simulink model "PMLSM_ControlCore_Block"  (R2026a)
settings: Solver=FixedStepDiscrete  StopTime=1  FixedStep=1e-4
values from neighbouring files (symbols this model uses):
  CPU_Clock = 200e6    (= 200000000)    [PMSLM_Init_Params_MBDL4.m]
  Current_Control_Mode = 2    [init_PMLSM_mil_test_params.m]
  DeadTime_Comp_Enable = 0    [init_PMLSM_mil_test_params.m]
  delay_N = 50    [PMSLM_Init_Params_MBDL4.m]
  DPCC_Ld_Factor = 1    [init_PMLSM_mil_test_params.m]
  DPCC_Lq_Factor = 1    [init_PMLSM_mil_test_params.m]
  DPCC_Psi_Factor = 1    [init_PMLSM_mil_test_params.m]
  DPCC_Rs_Factor = 1    [init_PMLSM_mil_test_params.m]
  DPICC_Ld_Factor = 1    [init_PMLSM_mil_test_params.m]
  DPICC_Lq_Factor = 1    [init_PMLSM_mil_test_params.m]
  Hold_Ticks = 30000    [PMSLM_Init_Params_MBDL4.m]
  Id_Init_Step = Id_Init_Target / Ramp_Ticks    (= 5e-05)    [PMSLM_Init_Params_MBDL4.m]
  Id_Init_Target = 0.5    [PMSLM_Init_Params_MBDL4.m]
  Id_Release_Ramp_Ticks = 2000    [PMSLM_Init_Params_MBDL4.m]
  Iq_fric_run = 0.05    [PMSLM_Init_Params_MBDL4.m]
  Iq_fric_start = 0.40    (= 0.4)    [PMSLM_Init_Params_MBDL4.m]
  Iq_int_limit = 0.10    (= 0.1)    [PMSLM_Init_Params_MBDL4.m]
  Kaw_d = Kaw_q    (= 0.2)    [PMSLM_Init_Params_MBDL4.m]
  Kaw_q = 0.2    [PMSLM_Init_Params_MBDL4.m]
  Kaw_s = 0.4    [PMSLM_Init_Params_MBDL4.m]
  Ki_ACR = ACR_Commissioning_Scale*Ki_ACR_Baseline    (= 2962.5)    [PMSLM_Init_Params_MBDL4.m]    (also in init_PMLSM_mil_test_params.m = Kp_ACR*PMLSM_Rs_ohm/PMLSM_Lq_H)
  Ki_ASR = 0.05    [PMSLM_Init_Params_MBDL4.m]
  Kp_ACR = ACR_Commissioning_Scale*Kp_ACR_Baseline    (= 2.18125)    [PMSLM_Init_Params_MBDL4.m]    (also in init_PMLSM_mil_test_params.m = PMLSM_Lq_H/(4*MIL_AUM3S4_Current_PI_xi^2*MIL_AUM3S4_Current_)
  Kp_ASR = 0.03    [PMSLM_Init_Params_MBDL4.m]
  Kp_pos = 5    [PMSLM_Init_Params_MBDL4.m]
  PICDO_Dhat_Limit_A = 3.0    (= 3)    [init_PMLSM_mil_test_params.m]
  PICDO_Kd = 0.25    [init_PMLSM_mil_test_params.m]
  PICDO_Kx = 1.0    (= 1)    [init_PMLSM_mil_test_params.m]
  PMLSM_deadtime_ratio = PMLSM_deadtime_s * PMLSM_pwm_freq_Hz    (= 0.01)    [init_PMLSM_plant_params.m]
  PMLSM_Ld_H = Ld    (= 0.001745)    [PMSLM_Init_Params_MBDL4.m]    (also in init_PMLSM_plant_params.m)
  PMLSM_Lq_H = Lq    (= 0.001745)    [PMSLM_Init_Params_MBDL4.m]    (also in init_PMLSM_plant_params.m)
  PMLSM_psi_f_Wb = flux    (= 0.141)    [PMSLM_Init_Params_MBDL4.m]    (also in init_PMLSM_plant_params.m)
  PMLSM_Rs_ohm = Rs    (= 2.37)    [PMSLM_Init_Params_MBDL4.m]    (also in init_PMLSM_plant_params.m)
  Pos_deadband = 0.02    [PMSLM_Init_Params_MBDL4.m]
  Ramp_Ticks = 10000    [PMSLM_Init_Params_MBDL4.m]
  Speed_Feedback_Mode = 1    [init_PMLSM_mil_test_params.m]
  Speed_loop_Iq_Limit = Iq_Limit    (= 0.3)    [PMSLM_Init_Params_MBDL4.m]
  Tau_e_mm = 60    [PMSLM_Init_Params_MBDL4.m]
  theta_align_const = 0    [PMSLM_Init_Params_MBDL4.m]
  Theta_Offset_Fine = Simulink.Parameter    [PMSLM_Init_Params_MBDL4.m]
  Ts = 1 / PWM_Freq    (= 0.0001)    [PMSLM_Init_Params_MBDL4.m]
  Ts_ACR = 1e-4    (= 0.0001)    [PMSLM_Init_Params_MBDL4.m]
  Ts_ASR = 1e-3    (= 0.001)    [PMSLM_Init_Params_MBDL4.m]
  Ts_DPICC = 1e-4    (= 0.0001)    [init_PMLSM_mil_test_params.m]
  Udc = 48    [PMSLM_Init_Params_MBDL4.m]    (also in init_PMLSM_mil_test_params.m)
  Uq_Zero_EN = 0：q 轴用正常 PI    [PMSLM_Init_Params_MBDL4.m]
  v_ff_eps = 0.5    [PMSLM_Init_Params_MBDL4.m]
  V_meas_max = 500    [PMSLM_Init_Params_MBDL4.m]
  v_meas_zero_eps = 0.5    [PMSLM_Init_Params_MBDL4.m]
  v_over_eps = 3    [PMSLM_Init_Params_MBDL4.m]
  V_pos_max_mmps = 10    [PMSLM_Init_Params_MBDL4.m]
  v_ref_max = 20    [PMSLM_Init_Params_MBDL4.m]
  v_ref_set_step_dn = v_ref_set_rate_dn * Ts    (= 0.005)    [PMSLM_Init_Params_MBDL4.m]
  v_ref_set_step_up = v_ref_set_rate_up * Ts    (= 0.005)    [PMSLM_Init_Params_MBDL4.m]
  v_ref_zero_eps = 0.2    [PMSLM_Init_Params_MBDL4.m]
  v_stick_off = 3.0    (= 3)    [PMSLM_Init_Params_MBDL4.m]
  v_stick_on = 1.0    (= 1)    [PMSLM_Init_Params_MBDL4.m]
  X_max_hard = 500    [PMSLM_Init_Params_MBDL4.m]
  X_max_soft = 470    [PMSLM_Init_Params_MBDL4.m]
  X_min_hard = -500    [PMSLM_Init_Params_MBDL4.m]
  X_min_soft = -470    [PMSLM_Init_Params_MBDL4.m]
libraries: hdlsllib x13, simulink x11, mcbeeMathTransformLib x2, mcbcontrolslib x1
(part 2 of 3)

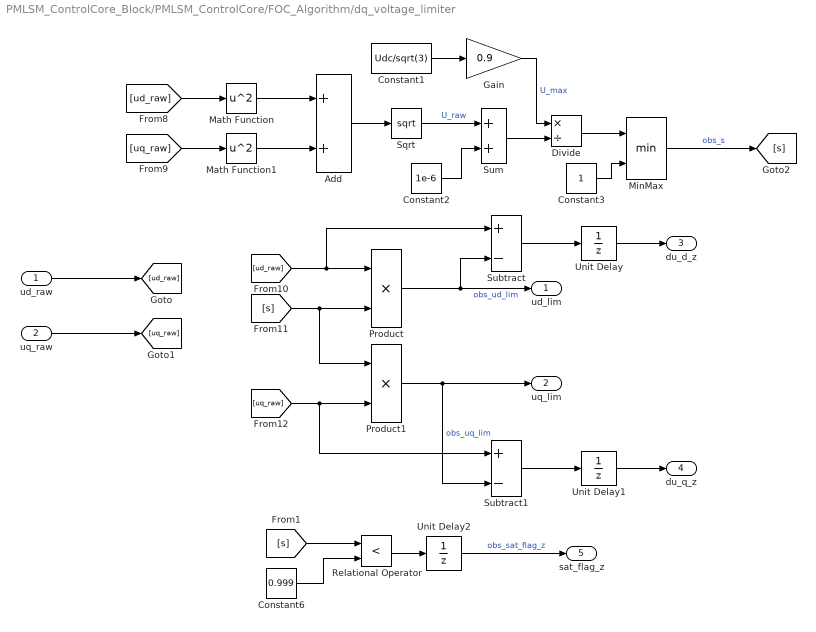
== system PMLSM_ControlCore_Block/PMLSM_ControlCore/FOC_Algorithm/dq_voltage_limiter ==
  ud_raw : Inport
  uq_raw : Inport  Port=2
  Add : Sum
  Constant1 : Constant  Value=Udc/sqrt(3)  OutDataTypeStr=double
  Constant2 : Constant  Value=1e-6  OutDataTypeStr=double
  Constant3 : Constant  OutDataTypeStr=double
  Constant6 : Constant  Value=0.999
  Divide : Product  Inputs=*/  OutDataTypeStr=double
  Gain : Gain  Gain=0.9  OutDataTypeStr=double
  Math Function : Math  Operator=square
  Math Function1 : Math  Operator=square
  MinMax : MinMax  Inputs=2
  Product : Product
  Product1 : Product  OutDataTypeStr=double
  Relational Operator : RelationalOperator  Operator=<  OutDataTypeStr=boolean  RndMeth=Simplest  InputSameDT=off
  Sqrt : Sqrt
  Subtract : Sum  Inputs=+-
  Subtract1 : Sum  Inputs=+-
  Sum : Sum
  Unit Delay : UnitDelay  SampleTime=-1
  Unit Delay1 : UnitDelay  SampleTime=-1
  Unit Delay2 : UnitDelay  SampleTime=-1
  ud_lim : Outport
  uq_lim : Outport  Port=2
  du_d_z : Outport  Port=3
  du_q_z : Outport  Port=4
  sat_flag_z : Outport  Port=5
  wires:
  Unit Delay2/1 -> sat_flag_z/1  "obs_sat_flag_z"
  Relational Operator/1 -> Unit Delay2/1
  [s] -> Relational Operator/1
  Constant6/1 -> Relational Operator/2
  Unit Delay1/1 -> du_q_z/1
  Unit Delay/1 -> du_d_z/1
  uq_raw/1 -> [uq_raw]
  ud_raw/1 -> [ud_raw]
  Subtract1/1 -> Unit Delay1/1
  Subtract/1 -> Unit Delay/1
  [uq_raw] -> Product1/2, Subtract1/1
  Product/1 -> ud_lim/1, Subtract/2  "obs_ud_lim"
  [ud_raw] -> Product/1, Subtract/1
  [s] -> Product/2, Product1/1
  Product1/1 -> Subtract1/2, uq_lim/1  "obs_uq_lim"
  MinMax/1 -> [s]  "obs_s"
  [ud_raw] -> Math Function/1
  [uq_raw] -> Math Function1/1
  Math Function/1 -> Add/1
  Math Function1/1 -> Add/2
  Sqrt/1 -> Sum/1  "U_raw"
  Gain/1 -> Divide/1  "U_max"
  Divide/1 -> MinMax/1
  Constant1/1 -> Gain/1
  Add/1 -> Sqrt/1
  Constant3/1 -> MinMax/2
  Constant2/1 -> Sum/2
  Sum/1 -> Divide/2

== system PMLSM_ControlCore_Block/PMLSM_ControlCore/Reference_Manager/v_ref_set_slew_limiter ==
  v_ref_set : Inport
  Add : Sum
  Saturation : Saturate  UpperLimit=v_ref_set_step_up  LowerLimit=-v_ref_set_step_dn
  Subtract : Sum  Inputs=+-
  v_ref_set_lim_z : UnitDelay  SampleTime=-1
  v_ref_set_limited : Outport
  wires:
  Add/1 -> v_ref_set_lim_z/1, v_ref_set_limited/1
  Subtract/1 -> Saturation/1
  Saturation/1 -> Add/1
  v_ref_set/1 -> Subtract/1
  v_ref_set_lim_z/1 -> Subtract/2, Add/2

== system PMLSM_ControlCore_Block/PMLSM_ControlCore/Triggered_Speed_loop/friction_compensation ==
  note: if start_mode == 1
      | 	iq_fric_mag = Iq_fric_start;
      | else
      | 	iq_fric_mag = Iq_fric_run;
      |
      | if ff_enable
      | 	iq_ff = iq_fric_mag * sign(v_ref);
      |  else
      | 	iq_ff = 0;
  v_ref : Inport
  abs_v_ref : Inport  Port=2
  abs_v_mmps : Inport  Port=3
  e_v : Inport  Port=4
  Compare To Constant1 : simulink/Logic and Bit Operations/Compare To Constant  relop=>  const=-v_over_eps  OutDataTypeStr=boolean
  Compare To Constant2 : simulink/Logic and Bit Operations/Compare To Constant  relop=>  const=v_ff_eps  OutDataTypeStr=boolean
  Constant1 : Constant  Value=Iq_fric_start
  Constant5 : Constant  Value=0
  Constant6 : Constant  Value=Iq_fric_run
  Gain : Gain  Gain=-1
  Logical Operator : Logic  AllPortsSameDT=off  OutDataTypeStr=boolean
  Product : Product
  Product1 : Product
  Product2 : Product
  Relay : Relay  OnSwitchValue=-v_stick_on  OffSwitchValue=-v_stick_off
  Sign : Signum
  Sign1 : Signum
  Switch : Switch  Criteria=u2 > Threshold  Threshold=0.5  SaturateOnIntegerOverflow=off  InputSameDT=off
  Switch2 : Switch  Criteria=u2 > Threshold  Threshold=0.5  SaturateOnIntegerOverflow=off  InputSameDT=off
  iq_ff : Outport
  wires:
  Gain/1 -> Relay/1
  Relay/1 -> Switch/2  "fric_start_mode"
  abs_v_mmps/1 -> Gain/1
  Logical Operator/1 -> Switch2/2  "ff_enable"
  Compare To Constant1/1 -> Logical Operator/2
  Compare To Constant2/1 -> Logical Operator/1
  Product2/1 -> Compare To Constant1/1
  e_v/1 -> Product2/2
  Product1/1 -> Switch/1
  Constant1/1 -> Product1/2
  Sign1/1 -> Product1/1
  Product/1 -> Switch/3
  Switch/1 -> Switch2/1
  Switch2/1 -> iq_ff/1  "iq_ff"
  abs_v_ref/1 -> Compare To Constant2/1
  Constant6/1 -> Product/2
  Constant5/1 -> Switch2/3
  Sign/1 -> Product/1, Product2/1
  v_ref/1 -> Sign1/1, Sign/1

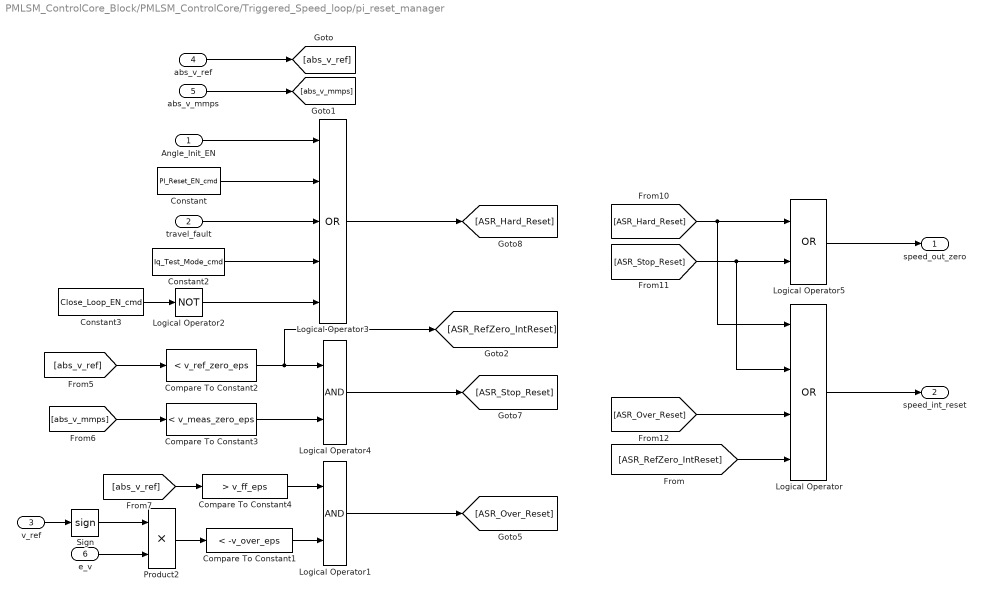
== system PMLSM_ControlCore_Block/PMLSM_ControlCore/Triggered_Speed_loop/pi_reset_manager ==
  Angle_Init_EN : Inport
  travel_fault : Inport  Port=2
  v_ref : Inport  Port=3
  abs_v_ref : Inport  Port=4
  abs_v_mmps : Inport  Port=5
  e_v : Inport  Port=6
  Compare To Constant1 : simulink/Logic and Bit Operations/Compare To Constant  relop=<  const=-v_over_eps  OutDataTypeStr=boolean
  Compare To Constant2 : simulink/Logic and Bit Operations/Compare To Constant  relop=<  const=v_ref_zero_eps  OutDataTypeStr=boolean
  Compare To Constant3 : simulink/Logic and Bit Operations/Compare To Constant  relop=<  const=v_meas_zero_eps  OutDataTypeStr=boolean
  Compare To Constant4 : simulink/Logic and Bit Operations/Compare To Constant  relop=>  const=v_ff_eps  OutDataTypeStr=boolean
  Constant : DataStoreRead  DataStoreName=PI_Reset_EN_cmd  IndexOptions=Index vector (dialog)  Indices=1  OutputSizes=1
  Constant2 : DataStoreRead  DataStoreName=Iq_Test_Mode_cmd  IndexOptions=Index vector (dialog)  Indices=1  OutputSizes=1
  Constant3 : DataStoreRead  DataStoreName=Close_Loop_EN_cmd  IndexOptions=Index vector (dialog)  Indices=1  OutputSizes=1
  Logical Operator : Logic  Operator=OR  Inputs=4  AllPortsSameDT=off  OutDataTypeStr=boolean
  Logical Operator1 : Logic  AllPortsSameDT=off  OutDataTypeStr=boolean
  Logical Operator2 : Logic  Operator=NOT  AllPortsSameDT=off  OutDataTypeStr=boolean
  Logical Operator3 : Logic  Operator=OR  Inputs=5  AllPortsSameDT=off  OutDataTypeStr=boolean
  Logical Operator4 : Logic  AllPortsSameDT=off  OutDataTypeStr=boolean
  Logical Operator5 : Logic  Operator=OR  AllPortsSameDT=off  OutDataTypeStr=boolean
  Product2 : Product
  Sign : Signum
  speed_out_zero : Outport
  speed_int_reset : Outport  Port=2
  wires:
  [ASR_RefZero_IntReset] -> Logical Operator/4
  Logical Operator1/1 -> [ASR_Over_Reset]
  Logical Operator/1 -> speed_int_reset/1
  [ASR_Over_Reset] -> Logical Operator/3
  [ASR_Hard_Reset] -> Logical Operator/1, Logical Operator5/1
  [ASR_Stop_Reset] -> Logical Operator/2, Logical Operator5/2
  Logical Operator4/1 -> [ASR_Stop_Reset]
  Logical Operator5/1 -> speed_out_zero/1
  Logical Operator3/1 -> [ASR_Hard_Reset]
  Compare To Constant3/1 -> Logical Operator4/2
  abs_v_mmps/1 -> [abs_v_mmps]
  abs_v_ref/1 -> [abs_v_ref]
  v_ref/1 -> Sign/1
  Angle_Init_EN/1 -> Logical Operator3/1
  Compare To Constant4/1 -> Logical Operator1/1
  Compare To Constant1/1 -> Logical Operator1/2
  Product2/1 -> Compare To Constant1/1
  Sign/1 -> Product2/1
  travel_fault/1 -> Logical Operator3/3
  e_v/1 -> Product2/2
  [abs_v_ref] -> Compare To Constant4/1
  [abs_v_mmps] -> Compare To Constant3/1
  Logical Operator2/1 -> Logical Operator3/5
  [abs_v_ref] -> Compare To Constant2/1
  Compare To Constant2/1 -> Logical Operator4/1, [ASR_RefZero_IntReset]
  Constant2/1 -> Logical Operator3/4
  Constant3/1 -> Logical Operator2/1
  Constant/1 -> Logical Operator3/2

== system PMLSM_ControlCore_Block/PMLSM_ControlCore/FOC_Algorithm/DPCC_Current_Controller/DPCC_DPICC_Select ==
  ud_dpcc : Inport
  uq_dpcc : Inport  Port=2
  ud_dpicc : Inport  Port=3
  uq_dpicc : Inport  Port=4
  dpicc_active : Inport  Port=5
  Current_Control_Mode : Inport  Port=6
  ud_pi : Inport  Port=7
  uq_pi : Inport  Port=8
  d_active_select : Switch  Threshold=0.5
  d_mode_select : Switch  Threshold=2.5
  q_active_select : Switch  Threshold=0.5
  q_mode_select : Switch  Threshold=2.5
  ud_selected : Outport
  uq_selected : Outport  Port=2
  wires:
  q_mode_select/1 -> uq_selected/1
  d_mode_select/1 -> ud_selected/1
  uq_dpcc/1 -> q_mode_select/3
  q_active_select/1 -> q_mode_select/1
  ud_dpcc/1 -> d_mode_select/3
  Current_Control_Mode/1 -> q_mode_select/2, d_mode_select/2
  d_active_select/1 -> d_mode_select/1
  uq_pi/1 -> q_active_select/3
  uq_dpicc/1 -> q_active_select/1
  ud_pi/1 -> d_active_select/3
  dpicc_active/1 -> d_active_select/2, q_active_select/2
  ud_dpicc/1 -> d_active_select/1

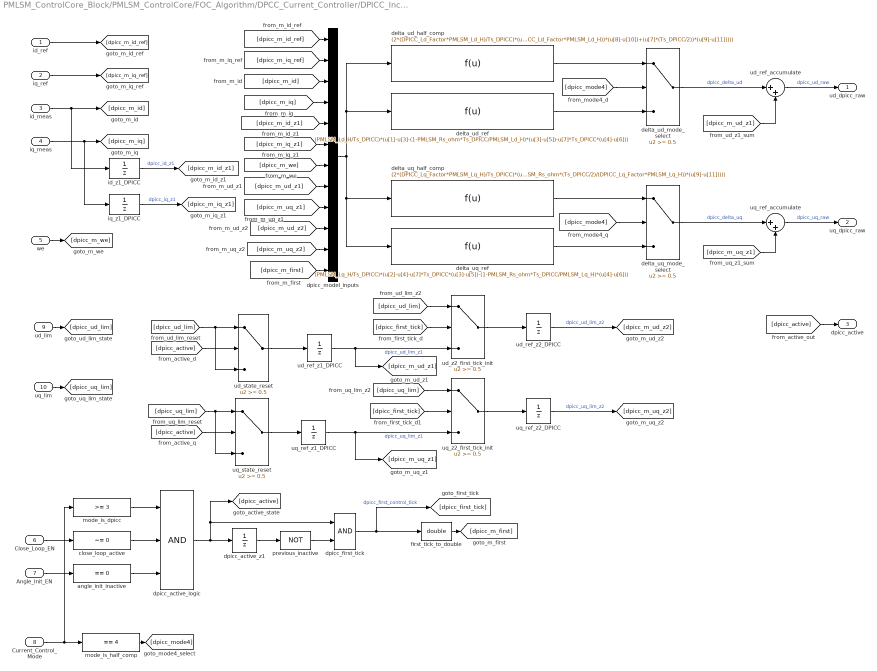
== system PMLSM_ControlCore_Block/PMLSM_ControlCore/FOC_Algorithm/DPCC_Current_Controller/DPICC_Incremental_Core ==
  id_ref : Inport
  iq_ref : Inport  Port=2
  id_meas : Inport  Port=3
  iq_meas : Inport  Port=4
  we : Inport  Port=5
  Close_Loop_EN : Inport  Port=6
  Angle_Init_EN : Inport  Port=7
  Current_Control_Mode : Inport  Port=8
  ud_lim : Inport  Port=9
  uq_lim : Inport  Port=10
  angle_init_inactive : hdlsllib/Logic and Bit Operations/Compare To Constant  relop===  const=0  OutDataTypeStr=boolean
  close_loop_active : hdlsllib/Logic and Bit Operations/Compare To Constant  relop=~=  const=0  OutDataTypeStr=boolean
  delta_ud_half_comp : Fcn  Expr=(2*(DPICC_Ld_Factor*PMLSM_Ld_H)/Ts_DPICC)*(u[1]-u[3]-(1-u[12])*(((1-PMLSM_Rs_ohm*(Ts_DPICC/2)/(DPICC_Ld_Factor*PMLSM_Ld_H))^2-(u[7]*(Ts_DPICC/2))^2)*(u[3]-u[5])+2*(1-PMLSM_Rs_ohm*(Ts_DPICC/2)/(DPICC_Ld_Factor*PMLSM_Ld_H))*(u[7]*(Ts_DPICC/2))*(u[4]-u[6])+(Ts_DPICC/2/(DPICC_Ld_Factor*PMLSM_Ld_H))*((1-PMLSM_Rs_ohm*(Ts_DPICC/2)/(DPICC_Ld_Factor*PMLSM_Ld_H))*(u[8]-u[10])+(u[7]*(Ts_DPICC/2))*(u[9]-u[11]))))
  delta_ud_mode_select : Switch  Threshold=0.5
  delta_ud_ref : Fcn  Expr=(PMLSM_Ld_H/Ts_DPICC)*(u[1]-u[3]-(1-PMLSM_Rs_ohm*Ts_DPICC/PMLSM_Ld_H)*(u[3]-u[5])-u[7]*Ts_DPICC*(u[4]-u[6]))
  delta_uq_half_comp : Fcn  Expr=(2*(DPICC_Lq_Factor*PMLSM_Lq_H)/Ts_DPICC)*(u[2]-u[4]-(1-u[12])*(-2*(1-PMLSM_Rs_ohm*(Ts_DPICC/2)/(DPICC_Lq_Factor*PMLSM_Lq_H))*(u[7]*(Ts_DPICC/2))*(u[3]-u[5])+((1-PMLSM_Rs_ohm*(Ts_DPICC/2)/(DPICC_Lq_Factor*PMLSM_Lq_H))^2-(u[7]*(Ts_DPICC/2))^2)*(u[4]-u[6])+(Ts_DPICC/2/(DPICC_Lq_Factor*PMLSM_Lq_H))*(-(u[7]*(Ts_DPICC/2))*(u[8]-u[10])+(1-PMLSM_Rs_ohm*(Ts_DPICC/2)/(DPICC_Lq_Factor*PMLSM_Lq_H))*(u[9]-u[11]))))
  delta_uq_mode_select : Switch  Threshold=0.5
  delta_uq_ref : Fcn  Expr=(PMLSM_Lq_H/Ts_DPICC)*(u[2]-u[4]-u[7]*Ts_DPICC*(u[3]-u[5])-(1-PMLSM_Rs_ohm*Ts_DPICC/PMLSM_Lq_H)*(u[4]-u[6]))
  dpicc_active_logic : Logic  Inputs=3
  dpicc_active_z1 : UnitDelay  SampleTime=-1
  dpicc_first_tick : Logic
  dpicc_model_inputs : Mux  Inputs=12
  first_tick_to_double : DataTypeConversion  OutDataTypeStr=double
  id_z1_DPICC : UnitDelay  SampleTime=-1  StateName=id_z1_DPICC
  iq_z1_DPICC : UnitDelay  SampleTime=-1  StateName=iq_z1_DPICC
  mode_is_dpicc : hdlsllib/Logic and Bit Operations/Compare To Constant  relop=>=  const=3  OutDataTypeStr=boolean
  mode_is_half_comp : hdlsllib/Logic and Bit Operations/Compare To Constant  relop===  const=4  OutDataTypeStr=boolean
  previous_inactive : Logic  Operator=NOT  Inputs=1
  ud_ref_accumulate : Sum  Inputs=|++
  ud_ref_z1_DPICC : UnitDelay  SampleTime=-1  StateName=ud_ref_z1_DPICC
  ud_ref_z2_DPICC : UnitDelay  SampleTime=-1
  ud_state_reset : Switch  Threshold=0.5
  ud_z2_first_tick_init : Switch  Threshold=0.5
  uq_ref_accumulate : Sum  Inputs=|++
  uq_ref_z1_DPICC : UnitDelay  SampleTime=-1  StateName=uq_ref_z1_DPICC
  uq_ref_z2_DPICC : UnitDelay  SampleTime=-1
  uq_state_reset : Switch  Threshold=0.5
  uq_z2_first_tick_init : Switch  Threshold=0.5
  ud_dpicc_raw : Outport
  uq_dpicc_raw : Outport  Port=2
  dpicc_active : Outport  Port=3
  wires:
  uq_ref_accumulate/1 -> uq_dpicc_raw/1  "dpicc_uq_raw"
  ud_ref_accumulate/1 -> ud_dpicc_raw/1  "dpicc_ud_raw"
  uq_ref_z1_DPICC/1 -> [dpicc_m_uq_z1], uq_z2_first_tick_init/3  "dpicc_uq_lim_z1"
  delta_uq_ref/1 -> delta_uq_mode_select/3
  ud_ref_z1_DPICC/1 -> [dpicc_m_ud_z1], ud_z2_first_tick_init/3  "dpicc_ud_lim_z1"
  delta_ud_ref/1 -> delta_ud_mode_select/3
  uq_state_reset/1 -> uq_ref_z1_DPICC/1
  ud_state_reset/1 -> ud_ref_z1_DPICC/1
  uq_lim/1 -> [dpicc_uq_lim]
  ud_lim/1 -> [dpicc_ud_lim]
  dpicc_model_inputs/1 -> delta_uq_half_comp/1, delta_uq_ref/1, delta_ud_half_comp/1, delta_ud_ref/1
  we/1 -> [dpicc_m_we]
  iq_z1_DPICC/1 -> [dpicc_m_iq_z1]  "dpicc_iq_z1"
  id_z1_DPICC/1 -> [dpicc_m_id_z1]  "dpicc_id_z1"
  iq_ref/1 -> [dpicc_m_iq_ref]
  id_ref/1 -> [dpicc_m_id_ref]
  iq_meas/1 -> [dpicc_m_iq], iq_z1_DPICC/1
  id_meas/1 -> [dpicc_m_id], id_z1_DPICC/1
  Current_Control_Mode/1 -> mode_is_half_comp/1, mode_is_dpicc/1
  Close_Loop_EN/1 -> close_loop_active/1
  Angle_Init_EN/1 -> angle_init_inactive/1
  mode_is_dpicc/1 -> dpicc_active_logic/1
  close_loop_active/1 -> dpicc_active_logic/2
  angle_init_inactive/1 -> dpicc_active_logic/3
  dpicc_active_logic/1 -> dpicc_first_tick/1, [dpicc_active], dpicc_active_z1/1
  dpicc_active_z1/1 -> previous_inactive/1
  previous_inactive/1 -> dpicc_first_tick/2
  delta_ud_half_comp/1 -> delta_ud_mode_select/1
  mode_is_half_comp/1 -> [dpicc_mode4]
  delta_uq_half_comp/1 -> delta_uq_mode_select/1
  delta_ud_mode_select/1 -> ud_ref_accumulate/1  "dpicc_delta_ud"
  delta_uq_mode_select/1 -> uq_ref_accumulate/1  "dpicc_delta_uq"
  dpicc_first_tick/1 -> first_tick_to_double/1, [dpicc_first_tick]  "dpicc_first_control_tick"
  ud_z2_first_tick_init/1 -> ud_ref_z2_DPICC/1
  ud_ref_z2_DPICC/1 -> [dpicc_m_ud_z2]  "dpicc_ud_lim_z2"
  uq_z2_first_tick_init/1 -> uq_ref_z2_DPICC/1
  uq_ref_z2_DPICC/1 -> [dpicc_m_uq_z2]  "dpicc_uq_lim_z2"
  first_tick_to_double/1 -> [dpicc_m_first]
  [dpicc_m_id_ref] -> dpicc_model_inputs/1
  [dpicc_m_iq_ref] -> dpicc_model_inputs/2
  [dpicc_m_id] -> dpicc_model_inputs/3
  [dpicc_m_iq] -> dpicc_model_inputs/4
  [dpicc_m_id_z1] -> dpicc_model_inputs/5
  [dpicc_m_iq_z1] -> dpicc_model_inputs/6
  [dpicc_m_we] -> dpicc_model_inputs/7
  [dpicc_m_ud_z1] -> dpicc_model_inputs/8
  [dpicc_m_uq_z1] -> dpicc_model_inputs/9
  [dpicc_m_ud_z2] -> dpicc_model_inputs/10
  [dpicc_m_uq_z2] -> dpicc_model_inputs/11
  [dpicc_m_first] -> dpicc_model_inputs/12
  [dpicc_mode4] -> delta_ud_mode_select/2
  [dpicc_mode4] -> delta_uq_mode_select/2
  [dpicc_first_tick] -> ud_z2_first_tick_init/2
  [dpicc_first_tick] -> uq_z2_first_tick_init/2
  [dpicc_active] -> ud_state_reset/2
  [dpicc_active] -> uq_state_reset/2
  [dpicc_active] -> dpicc_active/1
  [dpicc_ud_lim] -> ud_state_reset/1, ud_state_reset/3
  [dpicc_ud_lim] -> ud_z2_first_tick_init/1
  [dpicc_uq_lim] -> uq_state_reset/3, uq_state_reset/1
  [dpicc_uq_lim] -> uq_z2_first_tick_init/1
  [dpicc_m_ud_z1] -> ud_ref_accumulate/2
  [dpicc_m_uq_z1] -> uq_ref_accumulate/2

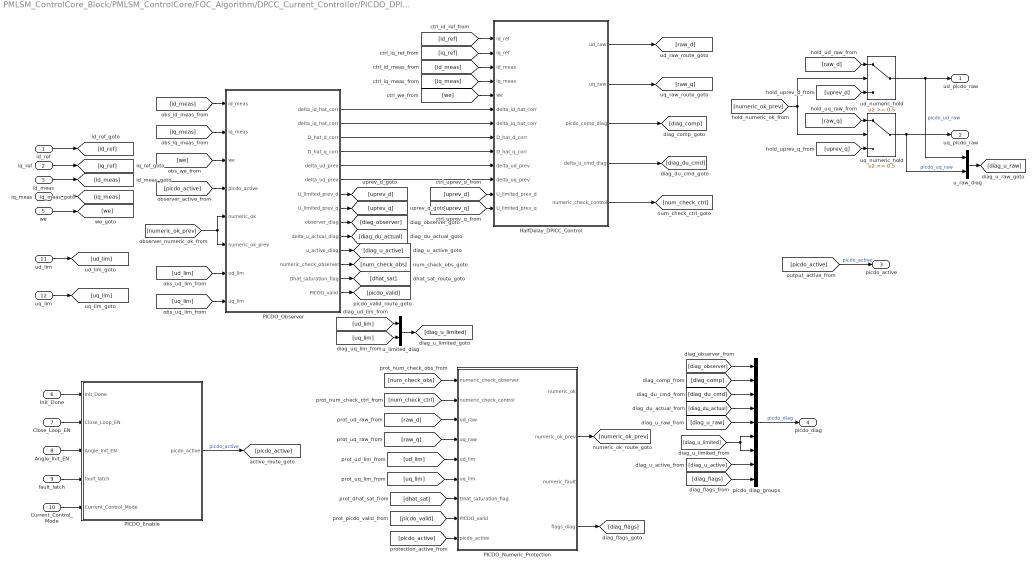
== system PMLSM_ControlCore_Block/PMLSM_ControlCore/FOC_Algorithm/DPCC_Current_Controller/PICDO_DPICC_Core ==
  id_ref : Inport
  iq_ref : Inport  Port=2
  id_meas : Inport  Port=3
  iq_meas : Inport  Port=4
  we : Inport  Port=5
  Init_Done : Inport  Port=6
  Close_Loop_EN : Inport  Port=7
  Angle_Init_EN : Inport  Port=8
  fault_latch : Inport  Port=9
  Current_Control_Mode : Inport  Port=10
  ud_lim : Inport  Port=11
  uq_lim : Inport  Port=12
  HalfDelay_DPICC_Control : Subsystem
  PICDO_Enable : Subsystem
  PICDO_Numeric_Protection : Subsystem
  PICDO_Observer : Subsystem
  picdo_diag_groups : Mux  Inputs=9
  u_limited_diag : Mux  Inputs=2
  u_raw_diag : Mux  Inputs=2
  ud_numeric_hold : Switch  Threshold=0.5
  uq_numeric_hold : Switch  Threshold=0.5
  ud_picdo_raw : Outport
  uq_picdo_raw : Outport  Port=2
  picdo_active : Outport  Port=3
  picdo_diag : Outport  Port=4
  wires:
  [numeric_ok_prev] -> uq_numeric_hold/2, ud_numeric_hold/2
  [numeric_ok_prev] -> PICDO_Observer/5(numeric_ok), PICDO_Observer/6(numeric_ok_prev)
  PICDO_Numeric_Protection/2(numeric_ok_prev) -> [numeric_ok_prev]
  [picdo_active] -> picdo_active/1  "picdo_active"
  [picdo_active] -> PICDO_Numeric_Protection/9(picdo_active)
  [picdo_active] -> PICDO_Observer/4(picdo_active)
  PICDO_Enable/1(picdo_active) -> [picdo_active]  "picdo_active"
  Init_Done/1 -> PICDO_Enable/1(Init_Done)
  Close_Loop_EN/1 -> PICDO_Enable/2(Close_Loop_EN)
  Angle_Init_EN/1 -> PICDO_Enable/3(Angle_Init_EN)
  fault_latch/1 -> PICDO_Enable/4(fault_latch)
  Current_Control_Mode/1 -> PICDO_Enable/5(Current_Control_Mode)
  id_meas/1 -> [id_meas]
  iq_meas/1 -> [iq_meas]
  we/1 -> [we]
  ud_lim/1 -> [ud_lim]
  uq_lim/1 -> [uq_lim]
  id_ref/1 -> [id_ref]
  iq_ref/1 -> [iq_ref]
  PICDO_Observer/1(delta_id_hat_corr) -> HalfDelay_DPICC_Control/6(delta_id_hat_corr)
  PICDO_Observer/2(delta_iq_hat_corr) -> HalfDelay_DPICC_Control/7(delta_iq_hat_corr)
  PICDO_Observer/3(D_hat_d_corr) -> HalfDelay_DPICC_Control/8(D_hat_d_corr)
  PICDO_Observer/4(D_hat_q_corr) -> HalfDelay_DPICC_Control/9(D_hat_q_corr)
  PICDO_Observer/5(delta_ud_prev) -> HalfDelay_DPICC_Control/10(delta_ud_prev)
  PICDO_Observer/6(delta_uq_prev) -> HalfDelay_DPICC_Control/11(delta_uq_prev)
  PICDO_Observer/7(U_limited_prev_d) -> [uprev_d]
  PICDO_Observer/8(U_limited_prev_q) -> [uprev_q]
  ud_numeric_hold/1 -> u_raw_diag/1, ud_picdo_raw/1  "picdo_ud_raw"
  uq_numeric_hold/1 -> uq_picdo_raw/1, u_raw_diag/2  "picdo_uq_raw"
  picdo_diag_groups/1 -> picdo_diag/1  "picdo_diag"
  PICDO_Observer/9(observer_diag) -> [diag_observer]
  HalfDelay_DPICC_Control/3(picdo_comp_diag) -> [diag_comp]
  HalfDelay_DPICC_Control/4(delta_u_cmd_diag) -> [diag_du_cmd]
  PICDO_Observer/10(delta_u_actual_diag) -> [diag_du_actual]
  u_raw_diag/1 -> [diag_u_raw]
  u_limited_diag/1 -> [diag_u_limited]
  PICDO_Observer/11(u_active_diag) -> [diag_u_active]
  PICDO_Numeric_Protection/4(flags_diag) -> [diag_flags]
  [diag_observer] -> picdo_diag_groups/1
  [diag_comp] -> picdo_diag_groups/2
  [diag_du_cmd] -> picdo_diag_groups/3
  [diag_du_actual] -> picdo_diag_groups/4
  [diag_u_raw] -> picdo_diag_groups/5
  [diag_u_limited] -> picdo_diag_groups/7, picdo_diag_groups/6
  [diag_u_active] -> picdo_diag_groups/8
  [diag_flags] -> picdo_diag_groups/9
  [uprev_d] -> ud_numeric_hold/3
  [uprev_q] -> uq_numeric_hold/3
  PICDO_Observer/12(numeric_check_observer) -> [num_check_obs]
  HalfDelay_DPICC_Control/5(numeric_check_control) -> [num_check_ctrl]
  HalfDelay_DPICC_Control/1(ud_raw) -> [raw_d]
  HalfDelay_DPICC_Control/2(uq_raw) -> [raw_q]
  PICDO_Observer/13(Dhat_saturation_flag) -> [dhat_sat]
  PICDO_Observer/14(PICDO_valid) -> [picdo_valid]
  [num_check_obs] -> PICDO_Numeric_Protection/1(numeric_check_observer)
  [num_check_ctrl] -> PICDO_Numeric_Protection/2(numeric_check_control)
  [raw_d] -> PICDO_Numeric_Protection/3(ud_raw)
  [raw_q] -> PICDO_Numeric_Protection/4(uq_raw)
  [dhat_sat] -> PICDO_Numeric_Protection/7(Dhat_saturation_flag)
  [picdo_valid] -> PICDO_Numeric_Protection/8(PICDO_valid)
  [raw_d] -> ud_numeric_hold/1
  [raw_q] -> uq_numeric_hold/1
  [id_ref] -> HalfDelay_DPICC_Control/1(id_ref)
  [iq_ref] -> HalfDelay_DPICC_Control/2(iq_ref)
  [id_meas] -> HalfDelay_DPICC_Control/3(id_meas)
  [iq_meas] -> HalfDelay_DPICC_Control/4(iq_meas)
  [we] -> HalfDelay_DPICC_Control/5(we)
  [id_meas] -> PICDO_Observer/1(id_meas)
  [iq_meas] -> PICDO_Observer/2(iq_meas)
  [we] -> PICDO_Observer/3(we)
  [ud_lim] -> PICDO_Observer/7(ud_lim)
  [uq_lim] -> PICDO_Observer/8(uq_lim)
  [ud_lim] -> PICDO_Numeric_Protection/5(ud_lim)
  [uq_lim] -> PICDO_Numeric_Protection/6(uq_lim)
  [ud_lim] -> u_limited_diag/1
  [uq_lim] -> u_limited_diag/2
  [uprev_d] -> HalfDelay_DPICC_Control/12(U_limited_prev_d)
  [uprev_q] -> HalfDelay_DPICC_Control/13(U_limited_prev_q)

== system PMLSM_ControlCore_Block/PMLSM_ControlCore/FOC_Algorithm/SVPWMG/Duty Calculate ==
  N : Inport
  T1 : Inport  Port=2
  T2 : Inport  Port=3
  Constant : Constant  Value=Ts
  Fcn : Fcn  Expr=(u[3]-u[1]-u[2])/4
  Fcn1 : Fcn  Expr=(u[3]+u[1]-u[2])/4
  Fcn2 : Fcn  Expr=(u[3]+u[2]+u[1])/4
  Gain : Gain  Gain=CPU_Clock
  Gain1 : Gain  Gain=CPU_Clock
  Gain2 : Gain  Gain=CPU_Clock
  Multiport Switch : MultiPortSwitch  Inputs=6  SaturateOnIntegerOverflow=off  InputSameDT=off
  Multiport Switch1 : MultiPortSwitch  Inputs=6  SaturateOnIntegerOverflow=off  InputSameDT=off
  Multiport Switch2 : MultiPortSwitch  Inputs=6  SaturateOnIntegerOverflow=off  InputSameDT=off
  Mux : Mux  Inputs=3
  Duty_U : Outport
  Duty_V : Outport  Port=2
  Duty_W : Outport  Port=3
  wires:
  Gain2/1 -> Duty_W/1  "DutyW"
  Gain1/1 -> Duty_V/1  "DutyV"
  Gain/1 -> Duty_U/1  "DutyU"
  N/1 -> Multiport Switch/1, Multiport Switch1/1, Multiport Switch2/1
  Fcn2/1 -> Multiport Switch2/4, Multiport Switch2/2, Multiport Switch1/7, Multiport Switch1/3, Multiport Switch/6, Multiport Switch/5
  Fcn1/1 -> Multiport Switch/2, Multiport Switch/7, Multiport Switch1/4, Multiport Switch2/6, Multiport Switch2/3, Multiport Switch1/5
  Fcn/1 -> Multiport Switch1/2, Multiport Switch2/7, Multiport Switch2/5, Multiport Switch1/6, Multiport Switch/4, Multiport Switch/3
  Multiport Switch/1 -> Gain/1
  Multiport Switch1/1 -> Gain1/1
  Multiport Switch2/1 -> Gain2/1
  T1/1 -> Mux/1
  T2/1 -> Mux/2
  Constant/1 -> Mux/3
  Mux/1 -> Fcn1/1, Fcn/1, Fcn2/1

== system PMLSM_ControlCore_Block/PMLSM_ControlCore/FOC_Algorithm/SVPWMG/Sector Caculate ==
  Ualpha : Inport
  Ubeta : Inport  Port=2
  B0 : Fcn  Expr=u[2]
  B1 : Fcn  Expr=u[1]*0.866-0.5*u[2]
  B2 : Fcn  Expr=-u[1]*0.866-u[2]*0.5
  Constant : Constant
  Constant1 : Constant  Value=0
  Mux : Mux  Inputs=2
  Mux1 : Mux  Inputs=3
  N : Fcn  Expr=4*u[3]+2*u[2]+u[1]
  Switch : Switch  Criteria=u2 > Threshold  SaturateOnIntegerOverflow=off  InputSameDT=off
  Switch1 : Switch  SaturateOnIntegerOverflow=off  InputSameDT=off
  Switch2 : Switch  Criteria=u2 > Threshold  SaturateOnIntegerOverflow=off  InputSameDT=off
  "N " : Outport  VectorParamsAs1DForOutWhenUnconnected=off
  wires:
  N/1 -> "N "/1  "N"
  Mux1/1 -> N/1
  Switch1/1 -> Mux1/2
  Constant1/1 -> Switch2/3, Switch1/3, Switch/3
  Constant/1 -> Switch1/1, Switch2/1, Switch/1
  B2/1 -> Switch2/2
  B1/1 -> Switch1/2
  B0/1 -> Switch/2
  Mux/1 -> B0/1, B1/1, B2/1
  Ubeta/1 -> Mux/2
  Ualpha/1 -> Mux/1
  Switch/1 -> Mux1/1
  Switch2/1 -> Mux1/3

== system PMLSM_ControlCore_Block/PMLSM_ControlCore/FOC_Algorithm/SVPWMG/T1T2 Calculate ==
  N : Inport
  X : Inport  Port=2
  Y : Inport  Port=3
  Z : Inport  Port=4
  Constant : Constant  Value=Ts
  Fcn : Fcn  Expr=u(3)-u(2)-u(1)
  Fcn1 : Fcn  Expr=u(1)*u(3)/(u(1)+u(2))
  Fcn2 : Fcn  Expr=u(2)*u(3)/(u(1)+u(2))
  Gain : Gain  Gain=-1
  Gain1 : Gain  Gain=-1
  Gain2 : Gain  Gain=-1
  Multiport Switch : MultiPortSwitch  Inputs=6  SaturateOnIntegerOverflow=off  InputSameDT=off
  Multiport Switch1 : MultiPortSwitch  Inputs=6  SaturateOnIntegerOverflow=off  InputSameDT=off
  Mux : Mux  Inputs=3
  Switch : Switch  SaturateOnIntegerOverflow=off  InputSameDT=off
  Switch1 : Switch  Criteria=u2 > Threshold  SaturateOnIntegerOverflow=off  InputSameDT=off
  T1 : Outport  VectorParamsAs1DForOutWhenUnconnected=off
  T2 : Outport  Port=2  VectorParamsAs1DForOutWhenUnconnected=off
  wires:
  Gain1/1 -> Multiport Switch/7, Multiport Switch1/6
  Gain2/1 -> Multiport Switch1/7, Multiport Switch/4
  Gain/1 -> Multiport Switch/5, Multiport Switch1/3
  X/1 -> Multiport Switch1/4, Multiport Switch/6, Gain/1
  Z/1 -> Gain2/1, Multiport Switch/2, Multiport Switch1/5
  Y/1 -> Gain1/1, Multiport Switch1/2, Multiport Switch/3
  N/1 -> Multiport Switch1/1, Multiport Switch/1
  Multiport Switch1/1 -> Mux/2, Switch1/1
  Multiport Switch/1 -> Mux/1, Switch/1
  Mux/1 -> Fcn2/1, Fcn/1, Fcn1/1
  Fcn/1 -> Switch1/2, Switch/2
  Fcn1/1 -> Switch/3
  Fcn2/1 -> Switch1/3
  Switch/1 -> T1/1  "T1"
  Switch1/1 -> T2/1  "T2"
  Constant/1 -> Mux/3

== system PMLSM_ControlCore_Block/PMLSM_ControlCore/FOC_Algorithm/SVPWMG/XYZ Calculate ==
  Ualpha : Inport
  Ubeta : Inport  Port=2
  Udc : Inport  Port=3
  Add : Sum
  Add1 : Sum  Inputs=+-
  Constant1 : Constant  Value=Ts
  Gain : Gain  Gain=3/2
  Gain1 : Gain  Gain=1.7321
  Gain2 : Gain  Gain=0.866
  Math Function : Math  Operator=reciprocal
  Product{,1..3} (4 alike) : Product
  X : Outport
  Y : Outport  Port=2
  Z : Outport  Port=3
  wires:
  Constant1/1 -> Product/1
  Product3/1 -> Y/1  "Y"
  Product2/1 -> Z/1  "Z"
  Add1/1 -> Product2/1
  Add/1 -> Product3/1
  Product1/1 -> X/1  "X"
  Gain/1 -> Add/2, Add1/2
  Gain2/1 -> Add1/1, Add/1
  Product/1 -> Product1/2, Product3/2, Product2/2
  Gain1/1 -> Product1/1
  Ubeta/1 -> Gain1/1, Gain2/1
  Math Function/1 -> Product/2
  Udc/1 -> Math Function/1
  Ualpha/1 -> Gain/1

== system PMLSM_ControlCore_Block/PMLSM_ControlCore/FOC_Algorithm/DPCC_Current_Controller/PICDO_DPICC_Core/HalfDelay_DPICC_Control ==
  id_ref : Inport
  iq_ref : Inport  Port=2
  id_meas : Inport  Port=3
  iq_meas : Inport  Port=4
  we : Inport  Port=5
  delta_id_hat_corr : Inport  Port=6
  delta_iq_hat_corr : Inport  Port=7
  D_hat_d_corr : Inport  Port=8
  D_hat_q_corr : Inport  Port=9
  delta_ud_prev : Inport  Port=10
  delta_uq_prev : Inport  Port=11
  U_limited_prev_d : Inport  Port=12
  U_limited_prev_q : Inport  Port=13
  U_picdo_comp_d : Gain  Gain=-(DPICC_Ld_Factor*PMLSM_Ld_H)/(Ts_DPICC/2)
  U_picdo_comp_q : Gain  Gain=-(DPICC_Lq_Factor*PMLSM_Lq_H)/(Ts_DPICC/2)
  control_inputs : Mux  Inputs=11
  delta_ud_cmd : Fcn  Expr=(2*(DPICC_Ld_Factor*PMLSM_Ld_H)/Ts_DPICC)*(u[1]-u[3]-(((1-PMLSM_Rs_ohm*(Ts_DPICC/2)/(DPICC_Ld_Factor*PMLSM_Ld_H))^2-(u[11]*(Ts_DPICC/2))^2)*u[5]+2*(1-PMLSM_Rs_ohm*(Ts_DPICC/2)/(DPICC_Ld_Factor*PMLSM_Ld_H))*(u[11]*(Ts_DPICC/2))*u[6]+((Ts_DPICC/2)/(DPICC_Ld_Factor*PMLSM_Ld_H))*((1-PMLSM_Rs_ohm*(Ts_DPICC/2)/(DPICC_Ld_Factor*PMLSM_Ld_H))*u[7]+(u[11]*(Ts_DPICC/2))*u[8]))-u[9])
  delta_uq_cmd : Fcn  Expr=(2*(DPICC_Lq_Factor*PMLSM_Lq_H)/Ts_DPICC)*(u[2]-u[4]-(-2*(1-PMLSM_Rs_ohm*(Ts_DPICC/2)/(DPICC_Lq_Factor*PMLSM_Lq_H))*(u[11]*(Ts_DPICC/2))*u[5]+((1-PMLSM_Rs_ohm*(Ts_DPICC/2)/(DPICC_Lq_Factor*PMLSM_Lq_H))^2-(u[11]*(Ts_DPICC/2))^2)*u[6]+((Ts_DPICC/2)/(DPICC_Lq_Factor*PMLSM_Lq_H))*(-(u[11]*(Ts_DPICC/2))*u[7]+(1-PMLSM_Rs_ohm*(Ts_DPICC/2)/(DPICC_Lq_Factor*PMLSM_Lq_H))*u[8]))-u[10])
  mux_delta_u_cmd : Mux  Inputs=2
  mux_numeric_check : Mux
  mux_picdo_comp : Mux  Inputs=2
  ud_raw_sum : Sum  Inputs=|++
  uq_raw_sum : Sum  Inputs=|++
  ud_raw : Outport
  uq_raw : Outport  Port=2
  picdo_comp_diag : Outport  Port=3
  delta_u_cmd_diag : Outport  Port=4
  numeric_check_control : Outport  Port=5
  wires:
  mux_numeric_check/1 -> numeric_check_control/1
  mux_delta_u_cmd/1 -> delta_u_cmd_diag/1
  mux_picdo_comp/1 -> picdo_comp_diag/1
  U_picdo_comp_q/1 -> mux_picdo_comp/2
  U_picdo_comp_d/1 -> mux_picdo_comp/1
  id_ref/1 -> control_inputs/1
  iq_ref/1 -> control_inputs/2
  id_meas/1 -> control_inputs/3
  iq_meas/1 -> control_inputs/4
  delta_id_hat_corr/1 -> control_inputs/5
  delta_iq_hat_corr/1 -> control_inputs/6
  delta_ud_prev/1 -> control_inputs/7
  delta_uq_prev/1 -> control_inputs/8
  D_hat_d_corr/1 -> U_picdo_comp_d/1, control_inputs/9
  D_hat_q_corr/1 -> control_inputs/10, U_picdo_comp_q/1
  we/1 -> control_inputs/11
  control_inputs/1 -> delta_ud_cmd/1, delta_uq_cmd/1
  U_limited_prev_d/1 -> ud_raw_sum/1
  delta_ud_cmd/1 -> mux_numeric_check/1, mux_delta_u_cmd/1, ud_raw_sum/2
  U_limited_prev_q/1 -> uq_raw_sum/1
  delta_uq_cmd/1 -> mux_numeric_check/2, uq_raw_sum/2, mux_delta_u_cmd/2
  ud_raw_sum/1 -> mux_numeric_check/3, ud_raw/1  "ud_raw"
  uq_raw_sum/1 -> mux_numeric_check/4, uq_raw/1  "uq_raw"

== system PMLSM_ControlCore_Block/PMLSM_ControlCore/FOC_Algorithm/DPCC_Current_Controller/PICDO_DPICC_Core/PICDO_Enable ==
  Init_Done : Inport
  Close_Loop_EN : Inport  Port=2
  Angle_Init_EN : Inport  Port=3
  fault_latch : Inport  Port=4
  Current_Control_Mode : Inport  Port=5
  angle_inactive : hdlsllib/Logic and Bit Operations/Compare To Constant  relop=<  const=0.5  OutDataTypeStr=boolean
  close_loop : hdlsllib/Logic and Bit Operations/Compare To Constant  relop=>=  const=0.5  OutDataTypeStr=boolean
  fault_inactive : hdlsllib/Logic and Bit Operations/Compare To Constant  relop===  const=0  OutDataTypeStr=boolean
  init_done : hdlsllib/Logic and Bit Operations/Compare To Constant  relop=>=  const=0.5  OutDataTypeStr=boolean
  mode_is_5 : hdlsllib/Logic and Bit Operations/Compare To Constant  relop===  const=5  OutDataTypeStr=boolean
  picdo_active_logic : Logic  Inputs=5  IconShape=distinctive
  picdo_active : Outport
  wires:
  Current_Control_Mode/1 -> mode_is_5/1
  Init_Done/1 -> init_done/1
  Close_Loop_EN/1 -> close_loop/1
  Angle_Init_EN/1 -> angle_inactive/1
  fault_latch/1 -> fault_inactive/1
  mode_is_5/1 -> picdo_active_logic/1
  init_done/1 -> picdo_active_logic/2
  close_loop/1 -> picdo_active_logic/3
  angle_inactive/1 -> picdo_active_logic/4
  fault_inactive/1 -> picdo_active_logic/5
  picdo_active_logic/1 -> picdo_active/1  "picdo_active"

== system PMLSM_ControlCore_Block/PMLSM_ControlCore/FOC_Algorithm/DPCC_Current_Controller/PICDO_DPICC_Core/PICDO_Numeric_Protection ==
  numeric_check_observer : Inport
  numeric_check_control : Inport  Port=2
  ud_raw : Inport  Port=3
  uq_raw : Inport  Port=4
  ud_lim : Inport  Port=5
  uq_lim : Inport  Port=6
  Dhat_saturation_flag : Inport  Port=7
  PICDO_valid : Inport  Port=8
  picdo_active : Inport  Port=9
  Dhat_sat_to_double : DataTypeConversion  OutDataTypeStr=double
  PICDO_valid_to_double : DataTypeConversion  OutDataTypeStr=double
  finite_check : MATLAB Function  TreatAsAtomicUnit=on
  mux_flags_diag : Mux  Inputs=5
  mux_numeric_inputs : Mux  Inputs=2
  numeric_fault_logic : Logic  Operator=NOT  IconShape=distinctive
  numeric_fault_to_double : DataTypeConversion  OutDataTypeStr=double
  numeric_ok_z1 : UnitDelay  InitialCondition=1  SampleTime=-1
  picdo_active_to_double : DataTypeConversion  OutDataTypeStr=double
  ud_saturated : hdlsllib/Logic and Bit Operations/Compare To Constant  relop=>  const=1e-8  OutDataTypeStr=boolean
  ud_saturation_abs : Abs
  ud_saturation_difference : Sum  Inputs=+-
  uq_saturated : hdlsllib/Logic and Bit Operations/Compare To Constant  relop=>  const=1e-8  OutDataTypeStr=boolean
  uq_saturation_abs : Abs
  uq_saturation_difference : Sum  Inputs=+-
  voltage_sat_to_double : DataTypeConversion  OutDataTypeStr=double
  voltage_saturation_flag : Logic  Operator=OR  IconShape=distinctive
  numeric_ok : Outport
  numeric_ok_prev : Outport  Port=2
  numeric_fault : Outport  Port=3
  flags_diag : Outport  Port=4
  wires:
  numeric_check_observer/1 -> mux_numeric_inputs/1
  numeric_check_control/1 -> mux_numeric_inputs/2
  mux_numeric_inputs/1 -> finite_check/1(u)
  finite_check/1(y) -> numeric_fault_logic/1, numeric_ok_z1/1, numeric_ok/1  "numeric_ok"
  numeric_ok_z1/1 -> numeric_ok_prev/1  "numeric_ok_prev"
  ud_raw/1 -> ud_saturation_difference/1
  ud_lim/1 -> ud_saturation_difference/2
  uq_raw/1 -> uq_saturation_difference/1
  uq_lim/1 -> uq_saturation_difference/2
  ud_saturation_difference/1 -> ud_saturation_abs/1
  uq_saturation_difference/1 -> uq_saturation_abs/1
  ud_saturation_abs/1 -> ud_saturated/1
  uq_saturation_abs/1 -> uq_saturated/1
  ud_saturated/1 -> voltage_saturation_flag/1
  uq_saturated/1 -> voltage_saturation_flag/2
  numeric_fault_logic/1 -> numeric_fault_to_double/1, numeric_fault/1  "PICDO_Numeric_Fault"
  voltage_saturation_flag/1 -> voltage_sat_to_double/1
  Dhat_saturation_flag/1 -> Dhat_sat_to_double/1
  PICDO_valid/1 -> PICDO_valid_to_double/1
  picdo_active/1 -> picdo_active_to_double/1
  voltage_sat_to_double/1 -> mux_flags_diag/1
  Dhat_sat_to_double/1 -> mux_flags_diag/2
  numeric_fault_to_double/1 -> mux_flags_diag/3
  PICDO_valid_to_double/1 -> mux_flags_diag/4
  picdo_active_to_double/1 -> mux_flags_diag/5
  mux_flags_diag/1 -> flags_diag/1

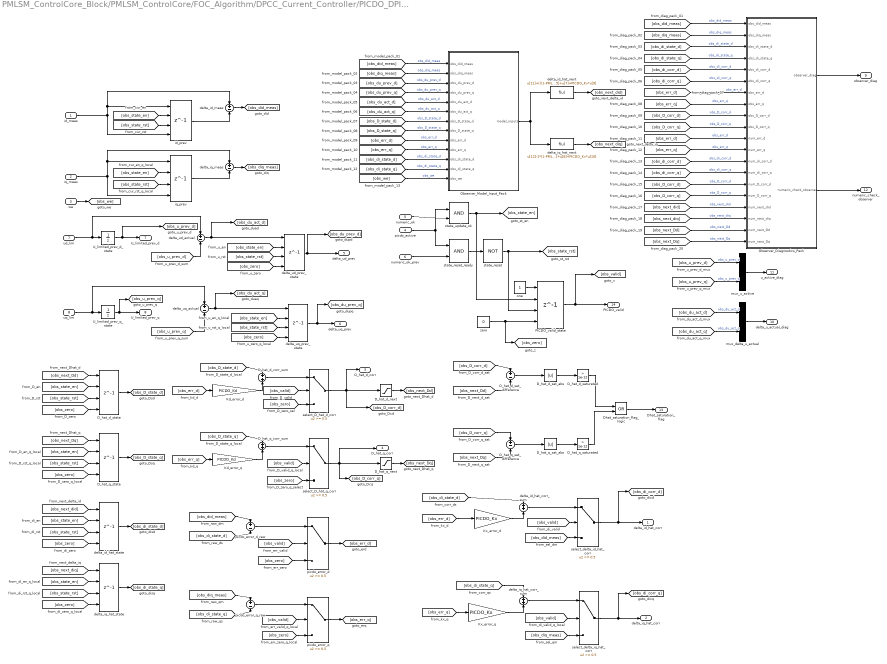
== system PMLSM_ControlCore_Block/PMLSM_ControlCore/FOC_Algorithm/DPCC_Current_Controller/PICDO_DPICC_Core/PICDO_Observer ==
  id_meas : Inport
  iq_meas : Inport  Port=2
  we : Inport  Port=3
  picdo_active : Inport  Port=4
  numeric_ok : Inport  Port=5
  numeric_ok_prev : Inport  Port=6
  ud_lim : Inport  Port=7
  uq_lim : Inport  Port=8
  D_hat_d_corr_sum : Sum
  D_hat_d_next : Saturate  UpperLimit=PICDO_Dhat_Limit_A  LowerLimit=-PICDO_Dhat_Limit_A
  D_hat_d_sat_abs : Abs
  D_hat_d_sat_difference : Sum  Inputs=+-
  D_hat_d_saturated : hdlsllib/Logic and Bit Operations/Compare To Constant  relop=>  const=1e-12  OutDataTypeStr=boolean
  D_hat_d_state : Delay  DelayLength=1  InitialConditionSource=Input port  ExternalReset=Level  ShowEnablePort=on  PreventDirectFeedthrough=on
      settings: InputPortMap=u0,e6,r5,p4
  D_hat_q_corr_sum : Sum
  D_hat_q_next : Saturate  UpperLimit=PICDO_Dhat_Limit_A  LowerLimit=-PICDO_Dhat_Limit_A
  D_hat_q_sat_abs : Abs
  D_hat_q_sat_difference : Sum  Inputs=+-
  D_hat_q_saturated : hdlsllib/Logic and Bit Operations/Compare To Constant  relop=>  const=1e-12  OutDataTypeStr=boolean
  D_hat_q_state : Delay  DelayLength=1  InitialConditionSource=Input port  ExternalReset=Level  ShowEnablePort=on  PreventDirectFeedthrough=on
      settings: InputPortMap=u0,e6,r5,p4
  Dhat_saturation_flag_logic : Logic  Operator=OR
  Kd_error_d : Gain  Gain=PICDO_Kd
  Kd_error_q : Gain  Gain=PICDO_Kd
  Kx_error_d : Gain  Gain=PICDO_Kx
  Kx_error_q : Gain  Gain=PICDO_Kx
  Observer_Diagnostics_Pack : Subsystem
  Observer_Model_Input_Pack : Subsystem
  PICDO_valid_state : Delay  DelayLength=1  InitialConditionSource=Input port  ExternalReset=Level  ShowEnablePort=on  PreventDirectFeedthrough=on
      settings: InputPortMap=u0,e6,r5,p4
  U_limited_prev_d_state : UnitDelay  SampleTime=-1
  U_limited_prev_q_state : UnitDelay  SampleTime=-1
  delta_id_hat_corr_sum : Sum
  delta_id_hat_next : Fcn  Expr=u[11]+(((1-PMLSM_Rs_ohm*(Ts_DPICC/2)/(DPICC_Ld_Factor*PMLSM_Ld_H))^2-(u[13]*(Ts_DPICC/2))^2)-1)*u[1]+2*(1-PMLSM_Rs_ohm*(Ts_DPICC/2)/(DPICC_Ld_Factor*PMLSM_Ld_H))*(u[13]*(Ts_DPICC/2))*u[2]+(Ts_DPICC/2)/(DPICC_Ld_Factor*PMLSM_Ld_H)*((1-PMLSM_Rs_ohm*(Ts_DPICC/2)/(DPICC_Ld_Factor*PMLSM_Ld_H))*u[3]+(u[13]*(Ts_DPICC/2))*u[4])+(Ts_DPICC/2)/(DPICC_Ld_Factor*PMLSM_Ld_H)*u[5]+u[7]+PICDO_Kx*u[9]
  delta_id_hat_state : Delay  DelayLength=1  InitialConditionSource=Input port  ExternalReset=Level  ShowEnablePort=on  PreventDirectFeedthrough=on
      settings: InputPortMap=u0,e6,r5,p4
  delta_id_meas : Sum  Inputs=+-
  delta_iq_hat_corr_sum : Sum
  delta_iq_hat_next : Fcn  Expr=u[12]-2*(1-PMLSM_Rs_ohm*(Ts_DPICC/2)/(DPICC_Lq_Factor*PMLSM_Lq_H))*(u[13]*(Ts_DPICC/2))*u[1]+(((1-PMLSM_Rs_ohm*(Ts_DPICC/2)/(DPICC_Lq_Factor*PMLSM_Lq_H))^2-(u[13]*(Ts_DPICC/2))^2)-1)*u[2]+(Ts_DPICC/2)/(DPICC_Lq_Factor*PMLSM_Lq_H)*(-(u[13]*(Ts_DPICC/2))*u[3]+(1-PMLSM_Rs_ohm*(Ts_DPICC/2)/(DPICC_Lq_Factor*PMLSM_Lq_H))*u[4])+(Ts_DPICC/2)/(DPICC_Lq_Factor*PMLSM_Lq_H)*u[6]+u[8]+PICDO_Kx*u[10]
  delta_iq_hat_state : Delay  DelayLength=1  InitialConditionSource=Input port  ExternalReset=Level  ShowEnablePort=on  PreventDirectFeedthrough=on
      settings: InputPortMap=u0,e6,r5,p4
  delta_iq_meas : Sum  Inputs=+-
  delta_ud_actual : Sum  Inputs=+-
  delta_ud_prev_state : Delay  DelayLength=1  InitialConditionSource=Input port  ExternalReset=Level  ShowEnablePort=on  PreventDirectFeedthrough=on
      settings: InputPortMap=u0,e6,r5,p4
  delta_uq_actual : Sum  Inputs=+-
  delta_uq_prev_state : Delay  DelayLength=1  InitialConditionSource=Input port  ExternalReset=Level  ShowEnablePort=on  PreventDirectFeedthrough=on
      settings: InputPortMap=u0,e6,r5,p4
  id_prev : Delay  DelayLength=1  InitialConditionSource=Input port  ExternalReset=Level  ShowEnablePort=on  PreventDirectFeedthrough=on
      settings: InputPortMap=u0,e6,r5,p4
  iq_prev : Delay  DelayLength=1  InitialConditionSource=Input port  ExternalReset=Level  ShowEnablePort=on  PreventDirectFeedthrough=on
      settings: InputPortMap=u0,e6,r5,p4
  mux_delta_u_actual : Mux  Inputs=2
  mux_u_active : Mux  Inputs=2
  one : Constant
  picdo_error_d : Switch  Threshold=0.5
  picdo_error_d_raw : Sum  Inputs=+-
  picdo_error_q : Switch  Threshold=0.5
  picdo_error_q_raw : Sum  Inputs=+-
  select_D_hat_d_corr : Switch  Threshold=0.5
  select_D_hat_q_corr : Switch  Threshold=0.5
  select_delta_id_hat_corr : Switch  Threshold=0.5
  select_delta_iq_hat_corr : Switch  Threshold=0.5
  state_reset : Logic  Operator=NOT  IconShape=distinctive
  state_reset_ready : Logic  IconShape=distinctive
  state_update_ok : Logic  IconShape=distinctive
  zero : Constant  Value=0
  delta_id_hat_corr : Outport
  delta_iq_hat_corr : Outport  Port=2
  D_hat_d_corr : Outport  Port=3
  D_hat_q_corr : Outport  Port=4
  delta_ud_prev : Outport  Port=5
  delta_uq_prev : Outport  Port=6
  U_limited_prev_d : Outport  Port=7
  U_limited_prev_q : Outport  Port=8
  observer_diag : Outport  Port=9
  delta_u_actual_diag : Outport  Port=10
  u_active_diag : Outport  Port=11
  numeric_check_observer : Outport  Port=12
  Dhat_saturation_flag : Outport  Port=13
  PICDO_valid : Outport  Port=14
  wires:
  [obs_next_Dq] -> D_hat_q_sat_difference/2
  [obs_D_corr_q] -> D_hat_q_sat_difference/1
  [obs_next_Dd] -> D_hat_d_sat_difference/2
  [obs_D_corr_d] -> D_hat_d_sat_difference/1
  [obs_D_state_q] -> D_hat_q_corr_sum/1
  [obs_D_state_d] -> D_hat_d_corr_sum/1
  we/1 -> [obs_we]
  select_delta_iq_hat_corr/1 -> [obs_di_corr_q], delta_iq_hat_corr/1
  select_delta_id_hat_corr/1 -> [obs_di_corr_d], delta_id_hat_corr/1
  select_D_hat_q_corr/1 -> D_hat_q_corr/1, D_hat_q_next/1, [obs_D_corr_q]
  select_D_hat_d_corr/1 -> D_hat_d_corr/1, D_hat_d_next/1, [obs_D_corr_d]
  D_hat_q_corr_sum/1 -> select_D_hat_q_corr/1
  D_hat_d_corr_sum/1 -> select_D_hat_d_corr/1
  delta_iq_hat_corr_sum/1 -> select_delta_iq_hat_corr/1
  delta_id_hat_corr_sum/1 -> select_delta_id_hat_corr/1
  D_hat_q_next/1 -> [obs_next_Dq]
  D_hat_d_next/1 -> [obs_next_Dd]
  Kd_error_q/1 -> D_hat_q_corr_sum/2
  D_hat_q_state/1 -> [obs_D_state_q]
  Kd_error_d/1 -> D_hat_d_corr_sum/2
  D_hat_d_state/1 -> [obs_D_state_d]
  Kx_error_q/1 -> delta_iq_hat_corr_sum/2
  Kx_error_d/1 -> delta_id_hat_corr_sum/2
  picdo_error_q/1 -> [obs_err_q]
  picdo_error_d/1 -> [obs_err_d]
  picdo_error_q_raw/1 -> picdo_error_q/1
  PICDO_valid_state/1 -> PICDO_valid/1, [obs_valid]
  picdo_error_d_raw/1 -> picdo_error_d/1
  delta_iq_hat_state/1 -> [obs_di_state_q]
  delta_iq_meas/1 -> [obs_diq_meas]
  delta_id_hat_state/1 -> [obs_di_state_d]
  delta_id_meas/1 -> [obs_did_meas]
  one/1 -> PICDO_valid_state/1
  zero/1 -> [obs_zero], PICDO_valid_state/4
  state_update_ok/1 -> PICDO_valid_state/2, [obs_state_en]
  picdo_active/1 -> state_reset_ready/1, state_update_ok/1
  numeric_ok/1 -> state_update_ok/2
  numeric_ok_prev/1 -> state_reset_ready/2
  state_reset_ready/1 -> state_reset/1
  state_reset/1 -> PICDO_valid_state/3, [obs_state_rst]
  [obs_next_did] -> delta_id_hat_state/1
  [obs_next_diq] -> delta_iq_hat_state/1
  [obs_next_Dd] -> D_hat_d_state/1
  [obs_next_Dq] -> D_hat_q_state/1
  [obs_state_en] -> D_hat_d_state/2
  [obs_state_rst] -> D_hat_d_state/3
  [obs_zero] -> D_hat_d_state/4
  [obs_state_en] -> delta_id_hat_state/2
  [obs_state_rst] -> delta_id_hat_state/3
  [obs_zero] -> delta_id_hat_state/4
  [obs_valid] -> picdo_error_d/2
  [obs_zero] -> picdo_error_d/3
  [obs_valid] -> select_delta_id_hat_corr/2
  [obs_valid] -> select_D_hat_d_corr/2
  [obs_zero] -> select_D_hat_d_corr/3
  [obs_did_meas] -> picdo_error_d_raw/1
  [obs_di_state_d] -> picdo_error_d_raw/2
  [obs_diq_meas] -> picdo_error_q_raw/1
  [obs_di_state_q] -> picdo_error_q_raw/2
  [obs_err_d] -> Kd_error_d/1
  [obs_err_q] -> Kd_error_q/1
  [obs_err_d] -> Kx_error_d/1
  [obs_err_q] -> Kx_error_q/1
  [obs_di_state_d] -> delta_id_hat_corr_sum/1
  [obs_di_state_q] -> delta_iq_hat_corr_sum/1
  [obs_did_meas] -> select_delta_id_hat_corr/3
  [obs_diq_meas] -> select_delta_iq_hat_corr/3
  [obs_zero] -> delta_ud_prev_state/4
  [obs_state_rst] -> delta_ud_prev_state/3
  [obs_state_en] -> delta_ud_prev_state/2
  [obs_state_rst] -> id_prev/3
  [obs_state_en] -> id_prev/2
  id_meas/1 -> id_prev/4, id_prev/1, delta_id_meas/1
  iq_meas/1 -> iq_prev/4, iq_prev/1, delta_iq_meas/1
  ud_lim/1 -> delta_ud_actual/1, U_limited_prev_d_state/1
  uq_lim/1 -> U_limited_prev_q_state/1, delta_uq_actual/1
  id_prev/1 -> delta_id_meas/2
  iq_prev/1 -> delta_iq_meas/2
  delta_ud_actual/1 -> [obs_du_act_d], delta_ud_prev_state/1
  delta_uq_actual/1 -> [obs_du_act_q], delta_uq_prev_state/1
  delta_ud_prev_state/1 -> [obs_du_prev_d], delta_ud_prev/1
  delta_uq_prev_state/1 -> delta_uq_prev/1, [obs_du_prev_q]
  U_limited_prev_d_state/1 -> [obs_u_prev_d], U_limited_prev_d/1
  U_limited_prev_q_state/1 -> [obs_u_prev_q], U_limited_prev_q/1
  [obs_state_en] -> iq_prev/2
  [obs_state_rst] -> iq_prev/3
  [obs_state_en] -> delta_uq_prev_state/2
  [obs_state_rst] -> delta_uq_prev_state/3
  [obs_zero] -> delta_uq_prev_state/4
  [obs_state_en] -> D_hat_q_state/2
  [obs_state_rst] -> D_hat_q_state/3
  [obs_zero] -> D_hat_q_state/4
  [obs_state_en] -> delta_iq_hat_state/2
  [obs_state_rst] -> delta_iq_hat_state/3
  [obs_zero] -> delta_iq_hat_state/4
  [obs_valid] -> select_D_hat_q_corr/2
  [obs_zero] -> select_D_hat_q_corr/3
  [obs_valid] -> picdo_error_q/2
  [obs_zero] -> picdo_error_q/3
  [obs_valid] -> select_delta_iq_hat_corr/2
  [obs_u_prev_d] -> delta_ud_actual/2
  [obs_u_prev_q] -> delta_uq_actual/2
  [obs_did_meas] -> Observer_Model_Input_Pack/1(obs_did_meas)  "obs_did_meas"
  [obs_diq_meas] -> Observer_Model_Input_Pack/2(obs_diq_meas)  "obs_diq_meas"
  [obs_du_prev_d] -> Observer_Model_Input_Pack/3(obs_du_prev_d)  "obs_du_prev_d"
  [obs_du_prev_q] -> Observer_Model_Input_Pack/4(obs_du_prev_q)  "obs_du_prev_q"
  [obs_du_act_d] -> Observer_Model_Input_Pack/5(obs_du_act_d)  "obs_du_act_d"
  [obs_du_act_q] -> Observer_Model_Input_Pack/6(obs_du_act_q)  "obs_du_act_q"
  [obs_D_state_d] -> Observer_Model_Input_Pack/7(obs_D_state_d)  "obs_D_state_d"
  [obs_D_state_q] -> Observer_Model_Input_Pack/8(obs_D_state_q)  "obs_D_state_q"
  [obs_err_d] -> Observer_Model_Input_Pack/9(obs_err_d)  "obs_err_d"
  [obs_err_q] -> Observer_Model_Input_Pack/10(obs_err_q)  "obs_err_q"
  [obs_di_state_d] -> Observer_Model_Input_Pack/11(obs_di_state_d)  "obs_di_state_d"
  [obs_di_state_q] -> Observer_Model_Input_Pack/12(obs_di_state_q)  "obs_di_state_q"
  [obs_we] -> Observer_Model_Input_Pack/13(obs_we)  "obs_we"
  [obs_did_meas] -> Observer_Diagnostics_Pack/1(obs_did_meas)  "obs_did_meas"
  [obs_diq_meas] -> Observer_Diagnostics_Pack/2(obs_diq_meas)  "obs_diq_meas"
  [obs_di_state_d] -> Observer_Diagnostics_Pack/3(obs_di_state_d)  "obs_di_state_d"
  [obs_di_state_q] -> Observer_Diagnostics_Pack/4(obs_di_state_q)  "obs_di_state_q"
  [obs_di_corr_d] -> Observer_Diagnostics_Pack/5(obs_di_corr_d)  "obs_di_corr_d"
  [obs_di_corr_q] -> Observer_Diagnostics_Pack/6(obs_di_corr_q)  "obs_di_corr_q"
  [obs_err_d] -> Observer_Diagnostics_Pack/7(obs_err_d)  "obs_err_d"
  [obs_err_q] -> Observer_Diagnostics_Pack/8(obs_err_q)  "obs_err_q"
  [obs_D_corr_d] -> Observer_Diagnostics_Pack/9(obs_D_corr_d)  "obs_D_corr_d"
  [obs_D_corr_q] -> Observer_Diagnostics_Pack/10(obs_D_corr_q)  "obs_D_corr_q"
  [obs_err_d] -> Observer_Diagnostics_Pack/11(num_err_d)  "obs_err_d"
  [obs_err_q] -> Observer_Diagnostics_Pack/12(num_err_q)  "obs_err_q"
  [obs_di_corr_d] -> Observer_Diagnostics_Pack/13(num_di_corr_d)  "obs_di_corr_d"
  [obs_di_corr_q] -> Observer_Diagnostics_Pack/14(num_di_corr_q)  "obs_di_corr_q"
  [obs_D_corr_d] -> Observer_Diagnostics_Pack/15(num_D_corr_d)  "obs_D_corr_d"
  [obs_D_corr_q] -> Observer_Diagnostics_Pack/16(num_D_corr_q)  "obs_D_corr_q"
  [obs_next_did] -> Observer_Diagnostics_Pack/17(num_next_did)  "obs_next_did"
  [obs_next_diq] -> Observer_Diagnostics_Pack/18(num_next_diq)  "obs_next_diq"
  [obs_next_Dd] -> Observer_Diagnostics_Pack/19(num_next_Dd)  "obs_next_Dd"
  [obs_next_Dq] -> Observer_Diagnostics_Pack/20(num_next_Dq)  "obs_next_Dq"
  Observer_Model_Input_Pack/1(model_inputs) -> delta_id_hat_next/1, delta_iq_hat_next/1
  delta_id_hat_next/1 -> [obs_next_did]
  delta_iq_hat_next/1 -> [obs_next_diq]
  Observer_Diagnostics_Pack/1(observer_diag) -> observer_diag/1
  Observer_Diagnostics_Pack/2(numeric_check_observer) -> numeric_check_observer/1
  D_hat_d_sat_difference/1 -> D_hat_d_sat_abs/1
  D_hat_d_sat_abs/1 -> D_hat_d_saturated/1
  D_hat_q_sat_difference/1 -> D_hat_q_sat_abs/1
  D_hat_q_sat_abs/1 -> D_hat_q_saturated/1
  D_hat_d_saturated/1 -> Dhat_saturation_flag_logic/1
  D_hat_q_saturated/1 -> Dhat_saturation_flag_logic/2
  Dhat_saturation_flag_logic/1 -> Dhat_saturation_flag/1
  [obs_u_prev_d] -> mux_u_active/1  "obs_u_prev_d"
  [obs_u_prev_q] -> mux_u_active/2  "obs_u_prev_q"
  [obs_du_act_d] -> mux_delta_u_actual/1  "obs_du_act_d"
  [obs_du_act_q] -> mux_delta_u_actual/2  "obs_du_act_q"
  mux_u_active/1 -> u_active_diag/1
  mux_delta_u_actual/1 -> delta_u_actual_diag/1
